simulink model "cognitwin_sdr_phy"  (R2025a)
settings: Solver=FixedStepDiscrete  StartTime=0.0  StopTime=SimStopTime  FixedStep=1/Fs  RelTol=1e-3
values from neighbouring files (symbols this model uses):
  ChannelGainIm = 0    [create_cognitwin_model.m]    (also in create_cognitwin_model_v3_backup.m)
  ChannelGainRe = 1    [create_cognitwin_model.m]    (also in create_cognitwin_model_v3_backup.m)
  InterferencePower = 0    [create_cognitwin_model.m]    (also in create_cognitwin_model_v3_backup.m)
  SNR_dB = 20    [create_cognitwin_model.m]    (also in create_cognitwin_model_v3_backup.m)
settings Model: Creator=dhire  LastModifiedBy=dhire

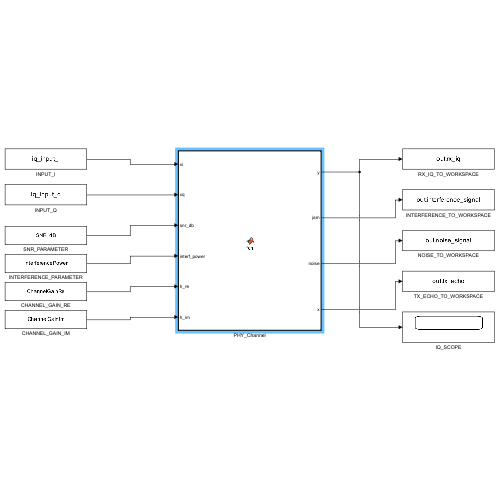
[thumbnail: Simulink's stored preview of the top-level diagram]
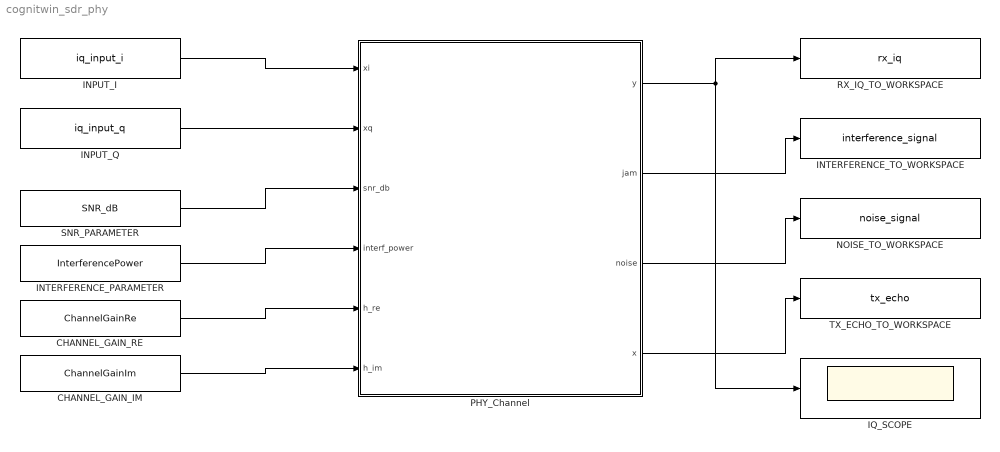
== system cognitwin_sdr_phy ==
  CHANNEL_GAIN_IM : Constant  Value=ChannelGainIm
  CHANNEL_GAIN_RE : Constant  Value=ChannelGainRe
  INPUT_I : FromWorkspace  VariableName=iq_input_i  Interpolate=off  OutputAfterFinalValue=Holding final value
  INPUT_Q : FromWorkspace  VariableName=iq_input_q  Interpolate=off  OutputAfterFinalValue=Holding final value
  INTERFERENCE_PARAMETER : Constant  Value=InterferencePower
  INTERFERENCE_TO_WORKSPACE : ToWorkspace  VariableName=interference_signal  SaveFormat=Structure With Time  SampleTime=-1
  IQ_SCOPE : Scope
      settings: ActiveDisplayYMinimum=-1.8795582889844731  ActiveDisplayYMaximum=1.8930181390179746
  NOISE_TO_WORKSPACE : ToWorkspace  VariableName=noise_signal  SaveFormat=Structure With Time  SampleTime=-1
  PHY_Channel : MATLAB Function  TreatAsAtomicUnit=on
  RX_IQ_TO_WORKSPACE : ToWorkspace  VariableName=rx_iq  SaveFormat=Structure With Time  SampleTime=-1
  SNR_PARAMETER : Constant  Value=SNR_dB
  TX_ECHO_TO_WORKSPACE : ToWorkspace  VariableName=tx_echo  SaveFormat=Structure With Time  SampleTime=-1
  wires:
  INPUT_I/1 -> PHY_Channel/1(xi)
  INPUT_Q/1 -> PHY_Channel/2(xq)
  SNR_PARAMETER/1 -> PHY_Channel/3(snr_db)
  INTERFERENCE_PARAMETER/1 -> PHY_Channel/4(interf_power)
  CHANNEL_GAIN_RE/1 -> PHY_Channel/5(h_re)
  CHANNEL_GAIN_IM/1 -> PHY_Channel/6(h_im)
  PHY_Channel/1(y) -> RX_IQ_TO_WORKSPACE/1, IQ_SCOPE/1
  PHY_Channel/2(jam) -> INTERFERENCE_TO_WORKSPACE/1
  PHY_Channel/3(noise) -> NOISE_TO_WORKSPACE/1
  PHY_Channel/4(x) -> TX_ECHO_TO_WORKSPACE/1

== matlab function cognitwin_sdr_phy/PHY_Channel ==
  data: xi input; y output; xq input; snr_db input; interf_power input; h_re input; h_im input; jam output; noise output; x output
function [y, jam, noise, x] = fcn(xi, xq, snr_db, interf_power, h_re, h_im)
x = complex(xi, xq);
h = complex(h_re, h_im);

noisePower = 10^(-snr_db/10);
noise = sqrt(noisePower/2) * complex(randn, randn);
jam   = sqrt(max(interf_power,0)/2) * complex(randn, randn);

y = h*x + jam + noise;
end
